simulink subsystem "imu_auto_zero"  (R2026a)
settings: Solver=VariableStepAuto
undefined symbols (not defined in the file): S
settings Model: Creator=rubystanton  LastModifiedBy=rubystanton

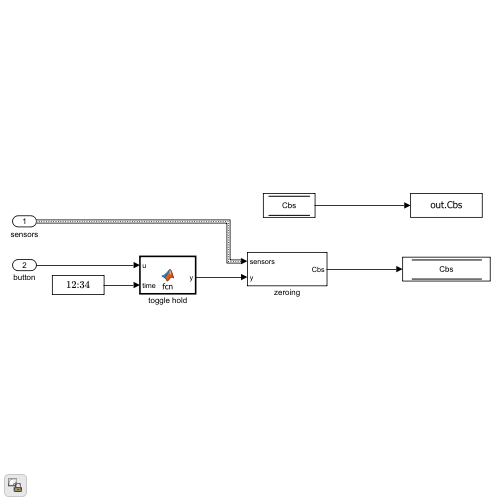
[thumbnail: Simulink's stored preview of the top-level diagram]
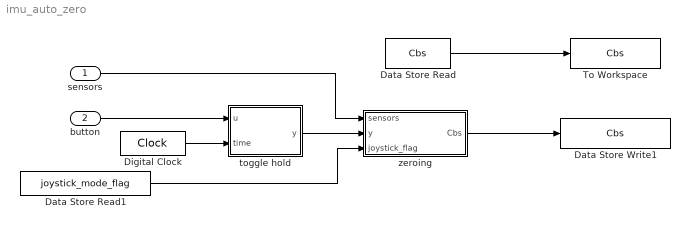
== system imu_auto_zero ==
  sensors : Inport
  button : Inport  Port=2
  Data Store Read : DataStoreRead  DataStoreName=Cbs  IndexOptions=Index vector (dialog)  Indices=1  OutputSizes=1
  Data Store Read1 : DataStoreRead  DataStoreName=joystick_mode_flag  IndexOptions=Index vector (dialog)  Indices=1  OutputSizes=1
  Data Store Write1 : DataStoreWrite  DataStoreName=Cbs  IndexOptions=Index vector (dialog)  Indices=1  OutputSizes=1
  Digital Clock : DigitalClock  SampleTime=S.dt_sim
  To Workspace : ToWorkspace  VariableName=Cbs  SaveFormat=Timeseries  SampleTime=-1
  toggle hold : MATLAB Function  TreatAsAtomicUnit=on
  zeroing : Subsystem
  wires:
  toggle hold/1(y) -> zeroing/2(y)
  Digital Clock/1 -> toggle hold/2(time)
  zeroing/1(Cbs) -> Data Store Write1/1
  Data Store Read/1 -> To Workspace/1
  sensors/1 -> zeroing/1(sensors)
  button/1 -> toggle hold/1(u)
  Data Store Read1/1 -> zeroing/3(joystick_flag)

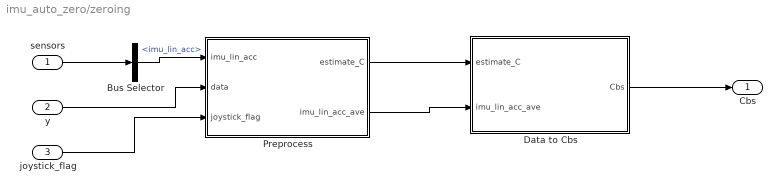
== system imu_auto_zero/zeroing ==
  sensors : Inport
  y : Inport  Port=2
  joystick_flag : Inport  Port=3
  Bus Selector : BusSelector  OutputSignals=imu_lin_acc
  Data to Cbs : MATLAB Function  TreatAsAtomicUnit=on
  Preprocess : MATLAB Function  TreatAsAtomicUnit=on
  Cbs : Outport
  wires:
  joystick_flag/1 -> Preprocess/3(joystick_flag)
  sensors/1 -> Bus Selector/1
  Bus Selector/1 -> Preprocess/1(imu_lin_acc)  "<imu_lin_acc>"
  Data to Cbs/1(Cbs) -> Cbs/1
  Preprocess/1(estimate_C) -> Data to Cbs/1(estimate_C)
  Preprocess/2(imu_lin_acc_ave) -> Data to Cbs/2(imu_lin_acc_ave)
  y/1 -> Preprocess/2(data)

== matlab function imu_auto_zero/toggle hold ==
  data: u input; y output; time input
function y = fcn(u, time)
%toggled true for 11 seconds after receiving a true button press
persistent zero_imu
persistent time_push
if isempty(zero_imu)
    zero_imu =false;
    time_push = -10;
end
if u == 1
    zero_imu = true;
    time_push = time;
end
if u~=1 && (time - time_push)>=11
    zero_imu = false;
end
y = zero_imu;

== matlab function imu_auto_zero/zeroing/Data to Cbs ==
  data: estimate_C input; imu_lin_acc_ave input; Cbs output; P parameter
function Cbs  = fcn(estimate_C,imu_lin_acc_ave,P)
% reevaluates zeroing rotation matrix
%
persistent Cbs_last;
if isempty(Cbs_last)
    Cbs_last = P.Sensors.imu.Cbimu_meas;
end
if estimate_C
    g_o = 9.80665;%[m/s^2]
    gi_ideal = [0;0;-g_o];
    %% Preprocessing
    options = optimoptions("fsolve",...
        Display="none",FunctionTolerance=1e-10,Algorithm="levenberg-marquardt");
    guess = [0*pi/180;0*pi/180;0*pi/180];
    %% Fsolve
    fun = @(x)rotation(x,gi_ideal,imu_lin_acc_ave);
    guess_new = fsolve(fun,guess,options);
    Cbs = eulToRotm(guess_new);
    Cbs_last = Cbs;
else
    Cbs = Cbs_last;
end
%% Helper function
function F = rotation(x,gi_ideal,sensor_read)
F = sqrt(((cos(x(2))*cos(x(3)) * gi_ideal(1)...
    +cos(x(2))*sin(x(3)) * gi_ideal(2)...
    -sin(x(2))*gi_ideal(3))-sensor_read(1))^2+...
    ((cos(x(1))*sin(x(2)) + sin(x(1))*sin(x(2))*cos(x(3)))*gi_ideal(1)...
    +(cos(x(1))*cos(x(3)) + sin(x(1)*sin(x(2))*sin(x(3))))*gi_ideal(2)...
    +sin(x(1))*cos(x(2))*gi_ideal(3)...
    - sensor_read(2))^2+...
    ((sin(x(1))*sin(x(3))+cos(x(1))*sin(x(2))*cos(x(3)))*gi_ideal(1)...
    +(-sin(x(1))*cos(x(3))+cos(x(1))*sin(x(2))*sin(x(3)))*gi_ideal(2)...
    +(cos(x(1))*cos(x(2)))*gi_ideal(3) ...
    -sensor_read(3))^2);
end
debug = Cbs(2);
end

== matlab function imu_auto_zero/zeroing/Preprocess ==
  data: estimate_C output; imu_lin_acc input; imu_lin_acc_ave output; data input; joystick_flag input
function [estimate_C,imu_lin_acc_ave] = fcn(imu_lin_acc, data,joystick_flag)
threshold = 10e3; %number of imu data points we're going off of
persistent averageing_index
persistent imu_lin_acc_stored 

if isempty(averageing_index)
    averageing_index = 0;
end    
if isempty(imu_lin_acc_stored)
    imu_lin_acc_stored = zeros(3,1,threshold); %indexes for 10s of data
end
averageing_index = averageing_index + 1;

if ~data
    averageing_index =0;
end


if joystick_flag&&(averageing_index < threshold && data)
    estimate_C = false;
    imu_lin_acc_stored(:,:,averageing_index) = imu_lin_acc(:);
    imu_lin_acc_ave = [0;0;-9.80665];
elseif joystick_flag&&averageing_index == threshold
    imu_lin_acc_stored(:,:,averageing_index) = imu_lin_acc(:);
    imu_lin_acc_ave = zeros(3,1);
    imu_lin_acc_ave(1) = mean(imu_lin_acc_stored(1,:,:));
    imu_lin_acc_ave(2) = mean(imu_lin_acc_stored(2,:,:));
    imu_lin_acc_ave(3) = mean(imu_lin_acc_stored(3,:,:));
    estimate_C = true;
else
    imu_lin_acc_ave = [0;0;-9.80665];
    estimate_C = false;
end
